simulink model "test_snap2"  (R2018a)
settings: Solver=VariableStepDiscrete  StartTime=0.0  StopTime=10.0  RelTol=1e-3
undefined symbols (not defined in the file): c
libraries: xbsIndex_r4 x21, xps_library x6, casper_library_misc x1
settings Model: Creator=jackh  LastModifiedBy=aisaacson
settings OptimizationCC: DefaultParameterBehavior=Inlined
settings DebuggingCC: LibraryContextMissingDiagnostic=warning
settings CodeAppCC: StateflowObjectComments=on

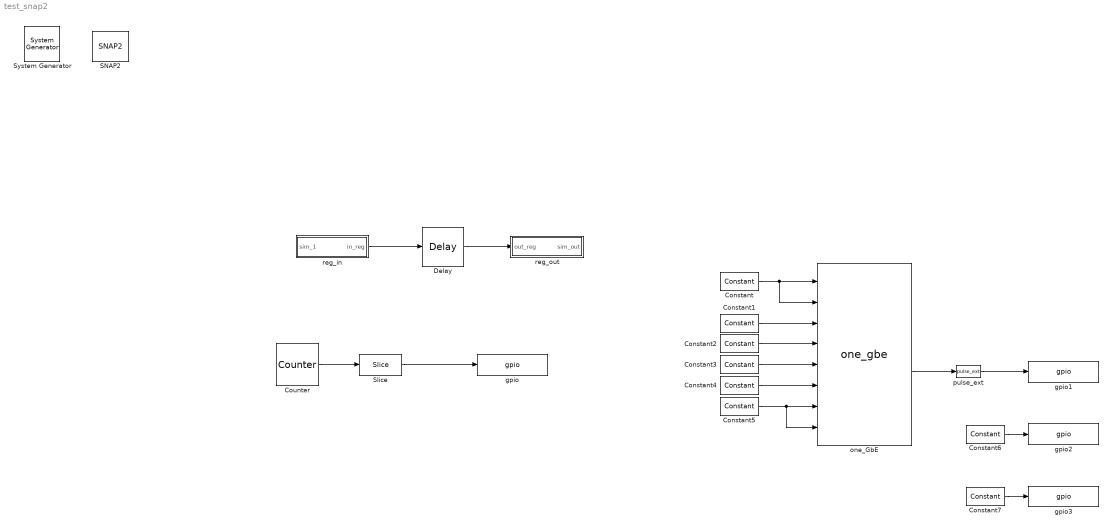
== system test_snap2 ==
  " System Generator" : xbsIndex_r4/ System Generator  Tag=genX  xilinxfamily=kintexu  part=xcku115  speed=-1-c  package=flvf1924  synthesis_tool=XST  clock_wrapper=Clock Enables  directory=/home/jasper/mlib_devel_2018/jasper_library/test_models/test_snap2/sysgen  proj_type=Vivado  Synth_file=Vivado Synthesis Defaults  Impl_file=Vivado Implementation Defaults  testbench=off  simulink_period=1  sysclk_period=10  dcm_input_clock_period=10  incr_netlist=off  trim_vbits=Everywhere in SubSystem  dbl_ovrd=According to Block Masks  core_generation=According to Block Masks  run_coregen=off  deprecated_control=off  eval_field=0  block_type=sysgen
  Constant{,2,5..7} (5 alike) : xbsIndex_r4/Constant  const=0  gui_display_data_type=Boolean  arith_type=Boolean  n_bits=16  bin_pt=14  preci_type=Single  exp_width=8  frac_width=24  explicit_period=on  period=1  equ=P=C  opselect=C  inp2=PCIN>>17  opr=+  inp1=P  carry=CIN  dbl_ovrd=off  block_type=constant
  Constant1 : xbsIndex_r4/Constant  const=0  gui_display_data_type=Fixed-point  arith_type=Unsigned  n_bits=8  bin_pt=0  preci_type=Single  exp_width=8  frac_width=24  explicit_period=on  period=1  equ=P=C  opselect=C  inp2=PCIN>>17  opr=+  inp1=P  carry=CIN  dbl_ovrd=off  block_type=constant
  Constant3 : xbsIndex_r4/Constant  const=0  gui_display_data_type=Fixed-point  arith_type=Unsigned  n_bits=32  bin_pt=0  preci_type=Single  exp_width=8  frac_width=24  explicit_period=on  period=1  equ=P=C  opselect=C  inp2=PCIN>>17  opr=+  inp1=P  carry=CIN  dbl_ovrd=off  block_type=constant
  Constant4 : xbsIndex_r4/Constant  const=0  gui_display_data_type=Fixed-point  arith_type=Unsigned  n_bits=16  bin_pt=0  preci_type=Single  exp_width=8  frac_width=24  explicit_period=on  period=1  equ=P=C  opselect=C  inp2=PCIN>>17  opr=+  inp1=P  carry=CIN  dbl_ovrd=off  block_type=constant
  Counter : xbsIndex_r4/Counter  cnt_type=Free Running  cnt_to=Inf  operation=Up  start_count=0  cnt_by_val=1  arith_type=Unsigned  n_bits=26  bin_pt=0  load_pin=off  rst=off  en=off  explicit_period=on  period=1  use_behavioral_HDL=off  implementation=Fabric  dbl_ovrd=off  block_type=counter
  Delay : xbsIndex_r4/Delay  rst=off  infoeditControl=Selection of Reset will increase slice count due to use of real FFs and instead of SRLs  en=off  latency=1  reg_retiming=off  dbl_ovrd=off  block_type=delay
  SNAP2 : xps_library/Platforms/SNAP2  Tag=xps:xsg  hw_sys=SNAP2:xcku115  clk_src=sys_clk  clk_rate=100  use_microblaze=on  sample_period=1  synthesis_tool=XST
      settings: SourceProductName=CASPER XPS Blockset
  Slice : xbsIndex_r4/Slice  nbits=1  boolean_output=on  mode=Upper Bit Location + Width  bit1=0  base1=MSB of Input  bit0=0  base0=LSB of Input  dbl_ovrd=off  block_type=slice
  gpio : xps_library/IO/gpio  Tag=xps:gpio  io_group_params_forwarded=on  io_group=ROACH:led  io_group_real=led  io_group_custom=0  io_dir=out  arith_type=Boolean  bitwidth=1  bin_pt=0  bit_index=0  sample_period=1  use_single_ended=off  use_ddr=off  reg_iob=on  reg_clk_phase=0  termination=None
      settings: SourceProductName=CASPER XPS Blockset
  gpio1 : xps_library/IO/gpio  Tag=xps:gpio  io_group_params_forwarded=on  io_group=ROACH:led  io_group_real=led  io_group_custom=0  io_dir=out  arith_type=Boolean  bitwidth=1  bin_pt=0  bit_index=1  sample_period=1  use_single_ended=off  use_ddr=off  reg_iob=on  reg_clk_phase=0  termination=None
      settings: SourceProductName=CASPER XPS Blockset
  gpio2 : xps_library/IO/gpio  Tag=xps:gpio  io_group_params_forwarded=on  io_group=ROACH:led  io_group_real=led  io_group_custom=0  io_dir=out  arith_type=Boolean  bitwidth=1  bin_pt=0  bit_index=2  sample_period=1  use_single_ended=off  use_ddr=off  reg_iob=on  reg_clk_phase=0  termination=None
      settings: SourceProductName=CASPER XPS Blockset
  gpio3 : xps_library/IO/gpio  Tag=xps:gpio  io_group_params_forwarded=on  io_group=ROACH:led  io_group_real=led  io_group_custom=0  io_dir=out  arith_type=Boolean  bitwidth=1  bin_pt=0  bit_index=3  sample_period=1  use_single_ended=off  use_ddr=off  reg_iob=on  reg_clk_phase=0  termination=None
      settings: SourceProductName=CASPER XPS Blockset
  one_GbE : xps_library/IO/one_gbe  Tag=xps:onegbe  local_en=on  dis_cpu_rx=off  dis_cpu_tx=off  cpu_promiscuous=on  local_mac=hex2dec('123456789abc')  local_ip=hex2dec('c0a8290a')  local_port=4321  local_gateway=1
      settings: SourceProductName=CASPER XPS Blockset
  pulse_ext : casper_library_misc/pulse_ext  pulse_len=2^26
      settings: SourceProductName=CASPER DSP Blockset
  reg_in : Subsystem  Tag=xps:sw_reg  AncestorBlock=xps_library/Memory/software_register  mask(swreg){io_dir=From Processor, io_delay=0, init_val=0, sample_period=1, names=reg, bitwidths=32, bin_pts=0, arith_types=0, sim_port=on, show_format=on}
      mask prompts: io_dir "I/O direction"; io_delay "I/O delay"; init_val "Initial Value"; sample_period "Sample period"; names "Bitfield names [msb...lsb]"; bitwidths "Bitfield widths"; bin_pts "Bitfield binary pts"; arith_types "Bitfield types, ufix=0, fix=1, bool=2"; sim_port "Provide sim input/output?"; show_format "Print format string?"
      mask help: A 32-bit software-accessible register. Can be divided into bitfields of varying widths and types using the fields in the block mask.
      mask init:
      | swreg_init(gcb)
      settings: AttributesFormatString=1input:uf32.0 = 32 bits
      mask TypeOptions io_dir: To Processor | From Processor
      mask Callback io_dir:
      | mask_enables = get_param(gcb, 'MaskEnables');
      | mask_names = get_param(gcb, 'MaskNames');
      | if strcmp(get_param(gcb, 'io_dir'), 'To Processor'),
      |     mask_enables{ismember(mask_names, 'sample_period')} = 'off';
      | else
      |     mask_enables{ismember(mask_names, 'sample_period')} = 'on';
      | end
      | set_param(gcb, 'MaskEnables', mask_enables);
      mask DialogControl ParameterTabVar0 Prompt: Setup
  reg_out : Subsystem  Tag=xps:sw_reg  AncestorBlock=xps_library/Memory/software_register  mask(swreg){io_dir=To Processor, io_delay=0, init_val=0, sample_period=1, names=reg, bitwidths=32, bin_pts=0, arith_types=0, sim_port=on, show_format=on}
      mask prompts: io_dir "I/O direction"; io_delay "I/O delay"; init_val "Initial Value"; sample_period "Sample period"; names "Bitfield names [msb...lsb]"; bitwidths "Bitfield widths"; bin_pts "Bitfield binary pts"; arith_types "Bitfield types, ufix=0, fix=1, bool=2"; sim_port "Provide sim input/output?"; show_format "Print format string?"
      mask help: A 32-bit software-accessible register. Can be divided into bitfields of varying widths and types using the fields in the block mask.
      mask init:
      | swreg_init(gcb)
      settings: AttributesFormatString=1output:uf32.0 = 32 bits
      mask TypeOptions io_dir: To Processor | From Processor
      mask Callback io_dir:
      | mask_enables = get_param(gcb, 'MaskEnables');
      | mask_names = get_param(gcb, 'MaskNames');
      | if strcmp(get_param(gcb, 'io_dir'), 'To Processor'),
      |     mask_enables{ismember(mask_names, 'sample_period')} = 'off';
      | else
      |     mask_enables{ismember(mask_names, 'sample_period')} = 'on';
      | end
      | set_param(gcb, 'MaskEnables', mask_enables);
      mask DialogControl ParameterTabVar0 Prompt: Setup
  wires:
  reg_in/1(in_reg) -> Delay/1
  Delay/1 -> reg_out/1(out_reg)
  Counter/1 -> Slice/1
  Slice/1 -> gpio/1
  Constant/1 -> one_GbE/2, one_GbE/1
  Constant1/1 -> one_GbE/3
  Constant2/1 -> one_GbE/4
  Constant3/1 -> one_GbE/5
  Constant4/1 -> one_GbE/6
  Constant5/1 -> one_GbE/8, one_GbE/7
  one_GbE/7 -> pulse_ext/1
  pulse_ext/1 -> gpio1/1
  Constant6/1 -> gpio2/1
  Constant7/1 -> gpio3/1

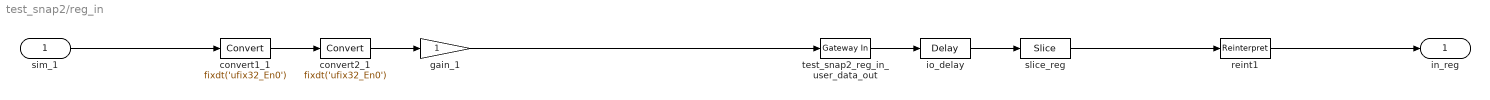
== system test_snap2/reg_in ==
  sim_1 : Inport
  convert1_1 : DataTypeConversion  OutDataTypeStr=fixdt('ufix32_En0')  LockScale=on
  convert2_1 : DataTypeConversion  OutDataTypeStr=fixdt('ufix32_En0')  ConvertRealWorld=Stored Integer (SI)  LockScale=on
  gain_1 : Gain
  io_delay : xbsIndex_r4/Delay  rst=off  infoeditControl=Selection of Reset will increase slice count due to use of real FFs and instead of SRLs  en=off  latency=0  reg_retiming=on  dbl_ovrd=off  block_type=delay
  reint1 : xbsIndex_r4/Reinterpret  force_arith_type=on  arith_type=Unsigned  force_bin_pt=on  bin_pt=0  block_type=reinterpret
  slice_reg : xbsIndex_r4/Slice  nbits=32  boolean_output=off  mode=Lower Bit Location + Width  bit1=0  base1=MSB of Input  bit0=0  base0=LSB of Input  dbl_ovrd=off  block_type=slice
  test_snap2_reg_in_user_data_out : xbsIndex_r4/Gateway In  gui_display_data_type=Fixed-point  arith_type=Unsigned  n_bits=32  bin_pt=0  preci_type=Single  exp_width=8  frac_width=24  rows=1  columns=1  quantization="Round  (unbiased: +/- Inf)"  overflow=Saturate  period=1  UseAsADC=off  ADCChannel='1'  interface=None  automatic_assignment=on  address_offset=hex2dec('00')  intf_name=''  intf_description=''  default_value=0  timing_constraint=None  locs_specified=off  LOCs={}  io_standard={}  inherit_from_input=off  hdl_port=on  dbl_ovrd=off  block_type=gatewayin
  in_reg : Outport
  wires:
  test_snap2_reg_in_user_data_out/1 -> io_delay/1
  sim_1/1 -> convert1_1/1
  convert1_1/1 -> convert2_1/1
  convert2_1/1 -> gain_1/1
  gain_1/1 -> test_snap2_reg_in_user_data_out/1
  io_delay/1 -> slice_reg/1
  slice_reg/1 -> reint1/1
  reint1/1 -> in_reg/1

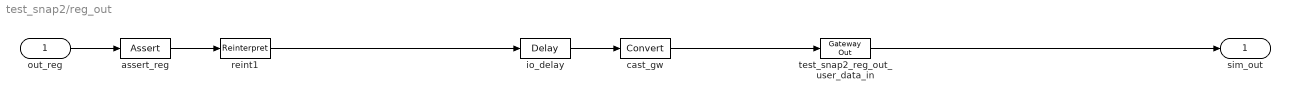
== system test_snap2/reg_out ==
  out_reg : Inport
  assert_reg : xbsIndex_r4/Assert  assert_type=on  type_source=Explicitly  gui_display_data_type=Fixed-point  arith_type=Unsigned  n_bits=32  bin_pt=0  preci_type=Single  exp_width=8  frac_width=24  assert_rate=off  rate_source=Explicitly  period=1  output_port=on  block_type=assert
  cast_gw : xbsIndex_r4/Convert  gui_display_data_type=Fixed-point  arith_type=Unsigned  n_bits=32  bin_pt=0  float_type=Single  exp_bits=8  fraction_bits=24  quantization=Truncate  overflow=Wrap  en=off  latency=1  pipeline=off  dbl_ovrd=off  block_type=convert
  io_delay : xbsIndex_r4/Delay  rst=off  infoeditControl=Selection of Reset will increase slice count due to use of real FFs and instead of SRLs  en=off  latency=0  reg_retiming=on  dbl_ovrd=off  block_type=delay
  reint1 : xbsIndex_r4/Reinterpret  force_arith_type=on  arith_type=Unsigned  force_bin_pt=on  bin_pt=0  block_type=reinterpret
  test_snap2_reg_out_user_data_in : xbsIndex_r4/Gateway Out  inherit_from_input=off  hdl_port=on  rows=1  columns=1  UseAsDAC=off  DACChannel='1'  interface=None  automatic_assignment=on  address_offset=hex2dec('00')  intf_name=''  intf_description=''  timing_constraint=None  locs_specified=off  LOCs={}  io_standard={}  block_type=gatewayout
  sim_out : Outport
  wires:
  io_delay/1 -> cast_gw/1
  cast_gw/1 -> test_snap2_reg_out_user_data_in/1
  test_snap2_reg_out_user_data_in/1 -> sim_out/1
  out_reg/1 -> assert_reg/1
  assert_reg/1 -> reint1/1
  reint1/1 -> io_delay/1
